simulink model "noise_gen"  (R2025b)
settings: Solver=FixedStepDiscrete  StartTime=0.0  StopTime=1  FixedStep=Ts  RelTol=1e-3
model workspace (MAT data in the model file):
  Ts = Simulink.Parameter
  Ts.Value = 0.0001
  Ts.Complexity = 'real'
  Ts.Dimensions = [1 1]
  Ts.CoderInfo.StorageClass = 'SimulinkGlobal'
  Ts.Description = 'Sample period [s] (= LabVIEW loop period)'
  Ts.DataType = 'auto'
  noise_std = Simulink.Parameter
  noise_std.Value = 0.2
  noise_std.Complexity = 'real'
  noise_std.Dimensions = [1 1]
  noise_std.CoderInfo.StorageClass = 'SimulinkGlobal'
  noise_std.Description = 'Noise standard deviation'
  noise_std.DataType = 'auto'
  sig_amp = Simulink.Parameter
  sig_amp.Value = 1
  sig_amp.Complexity = 'real'
  sig_amp.Dimensions = [1 1]
  sig_amp.CoderInfo.StorageClass = 'SimulinkGlobal'
  sig_amp.Description = 'Sine amplitude'
  sig_amp.DataType = 'auto'
  sig_freq = Simulink.Parameter
  sig_freq.Value = 10
  sig_freq.Complexity = 'real'
  sig_freq.Dimensions = [1 1]
  sig_freq.CoderInfo.StorageClass = 'SimulinkGlobal'
  sig_freq.Description = 'Sine frequency [Hz]'
  sig_freq.DataType = 'auto'
  sig_offset = Simulink.Parameter
  sig_offset.Value = 0
  sig_offset.Complexity = 'real'
  sig_offset.Dimensions = [1 1]
  sig_offset.CoderInfo.StorageClass = 'SimulinkGlobal'
  sig_offset.Description = 'DC offset'
  sig_offset.DataType = 'auto'
values from neighbouring files (symbols this model uses):
  Ts = max(Ts, 1e-6)    [signal_filter_core.m]
settings Model: Creator=REM2  LastModifiedBy=REM2
settings OptimizationCC: DefaultParameterBehavior=Inlined

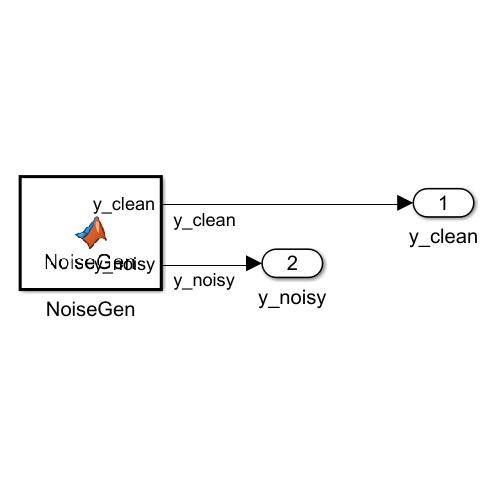
[thumbnail: Simulink's stored preview of the top-level diagram]
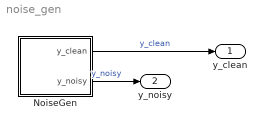
== system noise_gen ==
  NoiseGen : MATLAB Function  TreatAsAtomicUnit=on
  y_clean : Outport
  y_noisy : Outport  Port=2
  wires:
  NoiseGen/2(y_noisy) -> y_noisy/1  "y_noisy"
  NoiseGen/1(y_clean) -> y_clean/1  "y_clean"

== matlab function noise_gen/NoiseGen ==
  data: y_clean output; y_noisy output; Ts parameter; sig_amp parameter; sig_freq parameter; sig_offset parameter; noise_std parameter
function [y_clean, y_noisy] = NoiseGen(Ts, sig_amp, sig_freq, sig_offset, noise_std)
% Sine + white Gaussian noise. Inputs are tunable model-workspace parameters.
[y_clean, y_noisy] = noise_gen_core(Ts, sig_amp, sig_freq, sig_offset, noise_std);
